simulink model "mycpg"  (R2025b)
settings: Solver=VariableStepAuto  StartTime=0.0  StopTime=10.0  RelTol=1e-3
undefined symbols (not defined in the file or in its folder): np
settings Model: Creator=maria  LastModifiedBy=maria

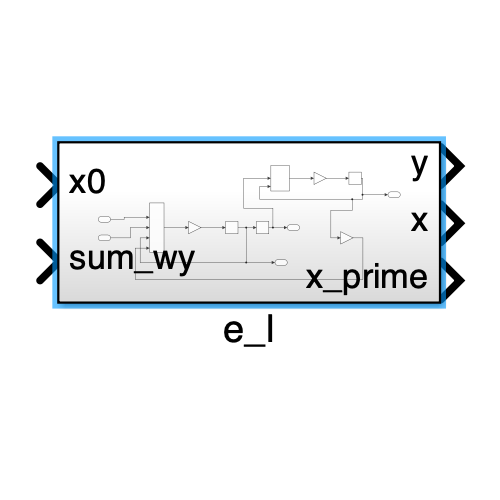
[thumbnail: Simulink's stored preview of the top-level diagram]
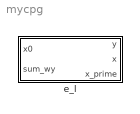
== system mycpg ==
  e_l : Subsystem

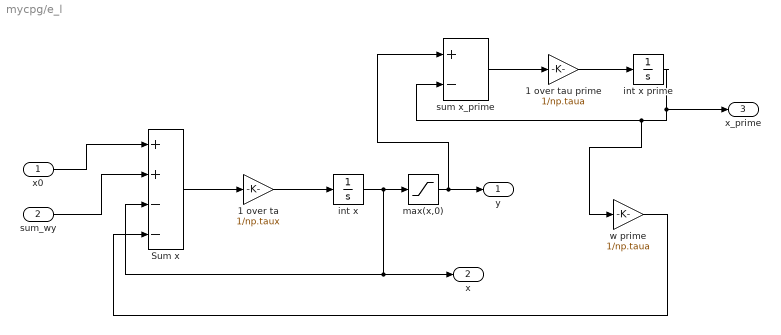
== system mycpg/e_l ==
  x0 : Inport
  sum_wy : Inport  Port=2
  1 over ta : Gain  Gain=1/np.taux
  1 over tau prime : Gain  Gain=1/np.taua
  Sum x : Sum  Inputs=|++--
  int x : Integrator
  int x prime : Integrator
  max(x,0) : Saturate  UpperLimit=inf  LowerLimit=0
  sum x_prime : Sum  Inputs=|+-
  w prime : Gain  Gain=1/np.taua
  y : Outport
  x : Outport  Port=2
  x_prime : Outport  Port=3
  wires:
  x0/1 -> Sum x/1
  sum_wy/1 -> Sum x/2
  Sum x/1 -> 1 over ta/1
  int x/1 -> x/1, Sum x/3, max(x,0)/1
  max(x,0)/1 -> sum x_prime/1, y/1
  1 over ta/1 -> int x/1
  sum x_prime/1 -> 1 over tau prime/1
  1 over tau prime/1 -> int x prime/1
  int x prime/1 -> x_prime/1, w prime/1, sum x_prime/2
  w prime/1 -> Sum x/4
